simulink model "Flowshield_Prototypefinal"  (R2025a)
settings: Solver=VariableStepAuto  StartTime=0.0  StopTime=100  RelTol=1e-3
settings Model: Creator=BCF05  LastModifiedBy=BCF05

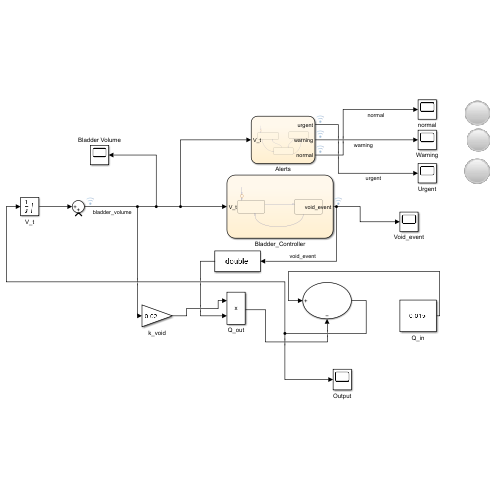
[thumbnail: Simulink's stored preview of the top-level diagram]
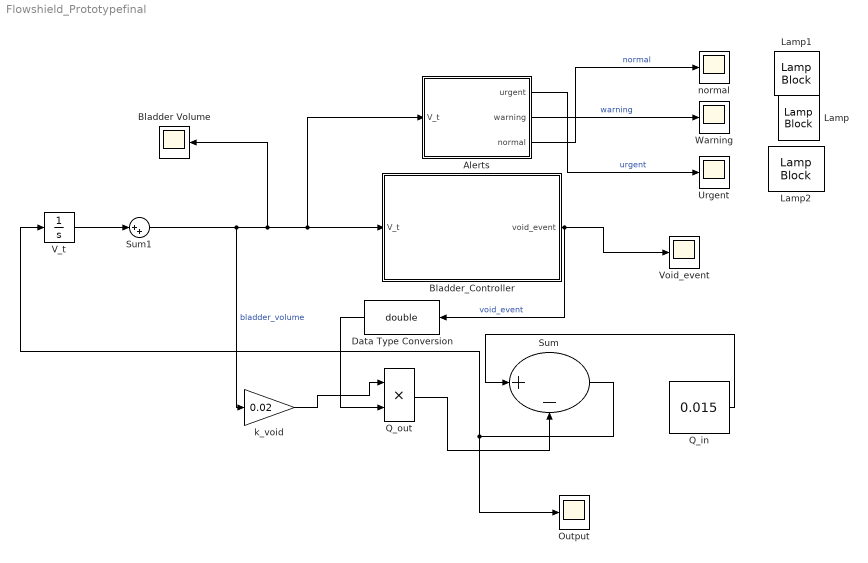
== system Flowshield_Prototypefinal ==
  Alerts : Stateflow chart  TreatAsAtomicUnit=on
  Bladder Volume : Scope
      settings: Title=Bladder Volume V(t) vs Time  ActiveDisplayYMinimum=299.81250000000017  ActiveDisplayYMaximum=301.68749999999847  YLabel=Bladder Volume, V(t) (mL)  DataLoggingVariableName=ScopeData4
  Bladder_Controller : Stateflow chart  TreatAsAtomicUnit=on
  Data Type Conversion : DataTypeConversion  OutDataTypeStr=double  SaturateOnIntegerOverflow=off  RndMeth=Floor
  Lamp : LampBlock  LabelPosition=Hide  DefaultColor=[192.0, 192.0, 192.0]
  Lamp1 : LampBlock  LabelPosition=Hide  DefaultColor=[192.0, 192.0, 192.0]
  Lamp2 : LampBlock  LabelPosition=Hide  DefaultColor=[192.0, 192.0, 192.0]
  Output : Scope
      settings: Title=Net Flow vs Time  ActiveDisplayYMinimum=0.0049999999999999992  ActiveDisplayYMaximum=0.025  YLabel=Net Flow  DataLoggingVariableName=ScopeData2
  Q_in : Constant  Value=0.015
  Q_out : Product  OutDataTypeStr=double  RndMeth=Round
  Sum : Sum  Inputs=|+-
  Sum1 : Sum  Inputs=|++
  Urgent : Scope
      settings: Title=Urgent Alert Activation vs Time  ActiveDisplayYMinimum=-0.13345195729537368  ActiveDisplayYMaximum=1.1790480427046266  YLabel=Urgent Alert Activation
  V_t : Integrator  InitialCondition=299  LimitOutput=on  UpperSaturationLimit=700  LowerSaturationLimit=0
  Void_event : Scope
      settings: Title=Void Event Signal Trigger vs Time  ActiveDisplayYMinimum=-1.3108070096855793  ActiveDisplayYMaximum=1.2417561153144219  YLabel=Void Event Signal Trigger
  Warning : Scope
      settings: Title=Warning Alert Activation vs Time  ActiveDisplayYMinimum=-0.12499999999999997  ActiveDisplayYMaximum=1.125  YLabel=Warning Alert Activation  DataLoggingVariableName=ScopeData3
  k_void : Gain  Gain=0.02  OutDataTypeStr=double
  normal : Scope
      settings: ActiveDisplayYMinimum=-0.12499999999999997  ActiveDisplayYMaximum=1.125  DataLoggingVariableName=ScopeData6
  wires:
  Bladder_Controller/1(void_event) -> Data Type Conversion/1, Void_event/1  "void_event"
  Alerts/1(urgent) -> Urgent/1  "urgent"
  Alerts/2(warning) -> Warning/1  "warning"
  Sum/1 -> V_t/1, Output/1
  Q_in/1 -> Sum/1
  Q_out/1 -> Sum/2
  k_void/1 -> Q_out/1
  Data Type Conversion/1 -> Q_out/2
  V_t/1 -> Sum1/1
  Sum1/1 -> k_void/1, Bladder Volume/1, Alerts/1(V_t), Bladder_Controller/1(V_t)  "bladder_volume"
  Alerts/3(normal) -> normal/1  "normal"

== stateflow chart Flowshield_Prototypefinal/Alerts ==
  state Urgent
    during: normal = false;
    warning = false; urgent = true;
  state Normal
    during: normal = true; warning = false;
    urgent = false;
  state Warning
    during: normal = false;
    warning = true; urgent = false;
  (default) -> (junction 14)
  (junction 14) -> Normal
  Urgent -> Warning : [V_t <= 550]
  Warning -> Urgent [order 2] : [V_t >=600]
  Normal -> Warning : [V_t >= 300]
  Warning -> Normal [order 1] : [V_t<=280]
  data: V_t input; urgent output boolean; warning output boolean; normal output

== stateflow chart Flowshield_Prototypefinal/Bladder_Controller ==
  state Voiding
    during:void_event = 1;
  state Filling
    during:
    void_event = 0;
  (default) -> (junction 67)
  (junction 67) -> Filling
  Filling -> Voiding : [V_t >= 600]
  Voiding -> Filling : [V_t <=150]
  data: V_t input; void_event output double
